simulink subsystem "Blade_Load_Scopes"  (R2025a)
settings: Solver=VariableStepAuto  StartTime=0.0  StopTime=10.0  RelTol=1e-3
Description:
  | Copyright 2025 The MathWorks, Inc.
settings Model: Creator=smiller  LastModifiedBy=smiller

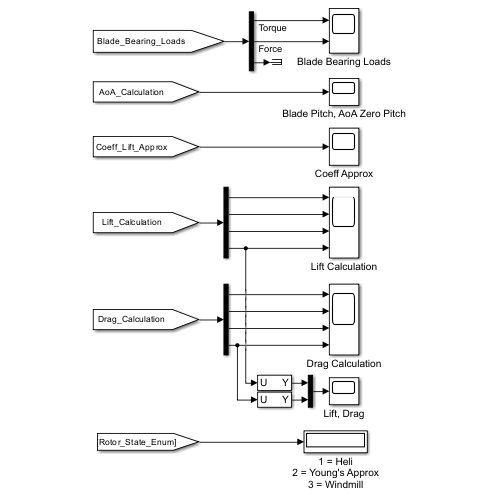
[thumbnail: Simulink's stored preview of the top-level diagram]
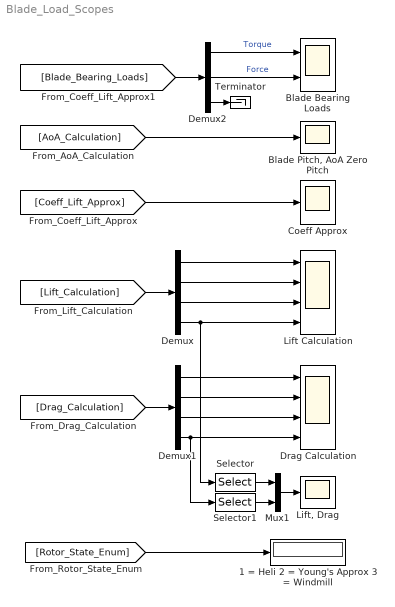
== system Blade_Load_Scopes ==
  1 = Heli 2 = Young's Approx 3 = Windmill : Display
      settings: RequirementInfo={} %GIDa_c5125553_7363_4e4d_9642_be499dd23722
  Blade Bearing Loads : Scope  NumInputPorts=2
      settings: RequirementInfo={} %GIDa_cca341eb_d75a_4e0c_b25a_746eb75cd85e  TimeSpan=80  ActiveDisplayYMinimum=-2.0E+6  ActiveDisplayYMaximum=4.0E+6
  "Blade Pitch, AoA Zero Pitch" : Scope
      settings: RequirementInfo={} %GIDa_62d70d3b_013a_4b35_b1bd_d079b9db9262  TimeSpan=400  ActiveDisplayYMinimum=0  ActiveDisplayYMaximum=100  DataLoggingVariableName=ScopeData2
  Coeff Approx : Scope
      settings: RequirementInfo={} %GIDa_bfba2eda_77e3_450e_983c_e1df138b043f  TimeSpan=400  ActiveDisplayYMinimum=-0.114  ActiveDisplayYMaximum=0.017941  DataLoggingVariableName=ScopeData3
  Demux : Demux  RequirementInfo={} %GIDa_0c665208_59a1_41c3_983f_3beea717cf69  Outputs=[1 3 3 3]
  Demux1 : Demux  RequirementInfo={} %GIDa_65decd13_130b_4a54_aafd_8e0067e3a22e  Outputs=[1 3 3 3]
  Demux2 : Demux  RequirementInfo={} %GIDa_f36dbe66_d067_4e79_a022_d680b3bf0805  Outputs=[3 3 12]
  Drag Calculation : Scope  NumInputPorts=4
      settings: RequirementInfo={} %GIDa_cc0f0612_5495_415f_a7ac_27df8da47285  TimeSpan=400  ActiveDisplayYMinimum=-2000  ActiveDisplayYMaximum=4000  DataLoggingVariableName=ScopeData4
  Lift Calculation : Scope  NumInputPorts=4
      settings: RequirementInfo={} %GIDa_92b9fd57_76b2_4162_b97d_cf5e43d5d8c9  TimeSpan=400  ActiveDisplayYMinimum=0  ActiveDisplayYMaximum=2000  DataLoggingVariableName=ScopeData5
  "Lift, Drag" : Scope
      settings: RequirementInfo={} %GIDa_72ddb878_8600_4a4f_bebc_31716d76e2c8  TimeSpan=160  ActiveDisplayYMinimum=-250.4352  ActiveDisplayYMaximum=408.3026
  Mux1 : Mux  RequirementInfo={} %GIDa_7ab843a4_22d6_48e9_9795_63091ad6056d  Inputs=2
  Selector : Selector  RequirementInfo={} %GIDa_4b5125f3_6226_4ae4_99e3_af6b2f6c7846  InputPortWidth=3  IndexOptions=Index vector (dialog)  Indices=[1]  OutputSizes=1
  Selector1 : Selector  RequirementInfo={} %GIDa_d518f4ce_1a78_4ff3_a718_281bedae5166  InputPortWidth=3  IndexOptions=Index vector (dialog)  Indices=[1 3]  OutputSizes=1
  Terminator : Terminator
      settings: RequirementInfo={} %GIDa_ca7f7885_18a7_48cf_bb1f_be42ffa68a6f
  wires:
  Demux2/2 -> Blade Bearing Loads/2  "Force"
  Demux/3 -> Lift Calculation/3
  Demux2/1 -> Blade Bearing Loads/1  "Torque"
  Demux1/4 -> Drag Calculation/4, Selector1/1
  Demux/1 -> Lift Calculation/1
  Demux2/3 -> Terminator/1
  Demux1/3 -> Drag Calculation/3
  Selector/1 -> Mux1/1
  [Rotor_State_Enum] -> 1 = Heli 2 = Young's Approx 3 = Windmill/1
  Selector1/1 -> Mux1/2
  [AoA_Calculation] -> "Blade Pitch, AoA Zero Pitch"/1
  [Lift_Calculation] -> Demux/1
  Demux/4 -> Lift Calculation/4, Selector/1
  [Coeff_Lift_Approx] -> Coeff Approx/1
  [Blade_Bearing_Loads] -> Demux2/1
  Mux1/1 -> "Lift, Drag"/1
  Demux1/1 -> Drag Calculation/1
  Demux/2 -> Lift Calculation/2
  Demux1/2 -> Drag Calculation/2
  [Drag_Calculation] -> Demux1/1
